simulink model "rlflight"  (R2024a)
settings: Solver=ode45  StartTime=0.0  StopTime=inf  RelTol=1e-3  EnableMultiTasking=on
libraries: instrumentlib x3, rllib x1
settings Model: Creator=The MathWorks, Inc.  LastModifiedBy=Administrator
settings SolverCC: AlgebraicLoopSolver=TrustRegion
settings DataIOCC: LimitDataPoints=on  SaveFormat=Array  SignalLoggingName=logsOut
settings OptimizationCC: ReuseModelBlockBuffer=off  ExpressionDepthLimit=2147483647  InitFltsAndDblsToZero=on  LifeSpan=inf
settings DebuggingCC: SaveWithParameterizedLinksMsg=none  UnderspecifiedInitializationDetection=Classic  MergeDetectMultiDrivingBlocksExec=none  SignalResolutionControl=TryResolveAllWithWarning  MultiTaskDSMMsg=warning  FcnCallInpInsideContextMsg=warning  UnconnectedInputMsg=warning  UnconnectedOutputMsg=warning  UnconnectedLineMsg=warning  AllowSymbolicDim=off  StateNameClashWarn=warning  SFUnexpectedBacktrackingDiag=warning  SFNoUnconditionalDefaultTransitionDiag=warning  SFExecutionAtInitializationDiag=none  ArithmeticOperatorsInVariantConditions=warning
settings HardwareCC: ProdBitPerPointer=32  ProdBitPerSizeT=32  ProdBitPerPtrDiffT=32  ProdLargestAtomicFloat=None  ProdIntDivRoundTo=Undefined  ProdEndianess=Unspecified  ProdWordSize=32  ProdHWDeviceType=Specified
settings ModelReferenceCC: EnableRefExpFcnMdlSchedulingChecks=on  PropagateSignalLabelsOutOfModel=off
settings SFSimCC: SimUseLocalCustomCode=off  CustomCodeUndefinedFunction=UseInterfaceOnly
settings RTWCC: RTWUseLocalCustomCode=off  GPUComputeCapability=3.5  DLArmComputeVersion=19.05
settings CodeAppCC: StateflowObjectComments=on
settings GRTTargetCC: TargetFcnLib=ansi_tfl_tmw.mat  TargetLangStandard=C89/C90 (ANSI)  CombineOutputUpdateFcns=off  GRTInterface=on
settings ConfigComp: CovMetricSettings=dw  CovSaveCumulativeToWorkspaceVar=on  CovSaveSingleToWorkspaceVar=on  CovExternalEMLEnable=off

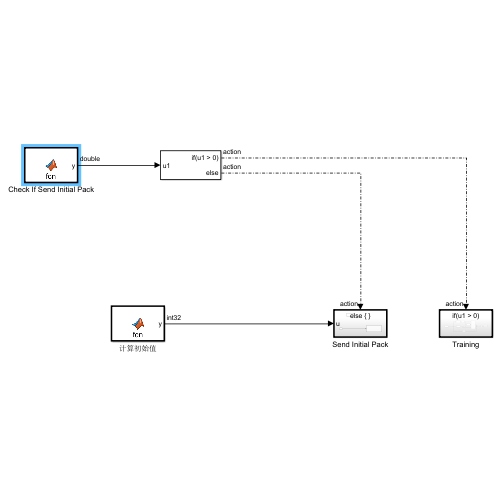
[thumbnail: Simulink's stored preview of the top-level diagram]
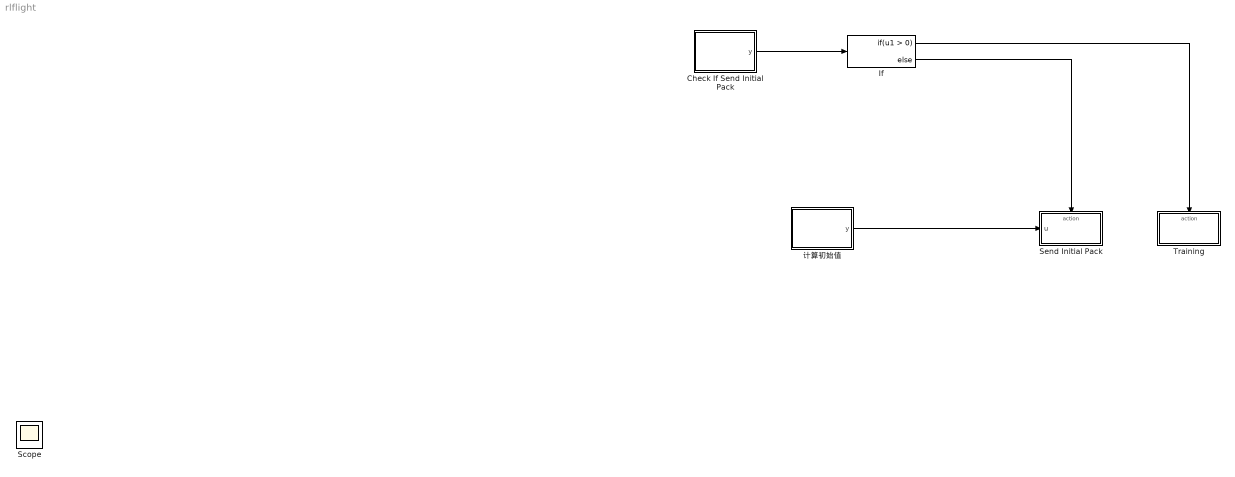
== system rlflight ==
  Check If Send Initial Pack : MATLAB Function  TreatAsAtomicUnit=on
  If : If
  Send Initial Pack : Subsystem  TreatAsAtomicUnit=on
  Training : Subsystem  TreatAsAtomicUnit=on
  计算初始值 : MATLAB Function  TreatAsAtomicUnit=on
  Scope : Scope
  wires:
  Check If Send Initial Pack/1(y) -> If/1
  If/2 -> Send Initial Pack/Action
  If/1 -> Training/Action
  计算初始值/1(y) -> Send Initial Pack/1(u)

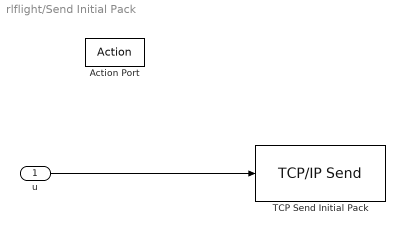
== system rlflight/Send Initial Pack ==
  u : Inport
  Action Port : ActionPort  ActionPortLabel=else
  TCP Send Initial Pack : instrumentlib/TCP//IP Send  Priority=1  Host=10.119.13.38  Port=1000  ByteOrder=little-endian  EnableBlockingMode=on  Timeout=5  TransferDelay=on  SimulateUsing=Interpreted execution
  wires:
  u/1 -> TCP Send Initial Pack/1

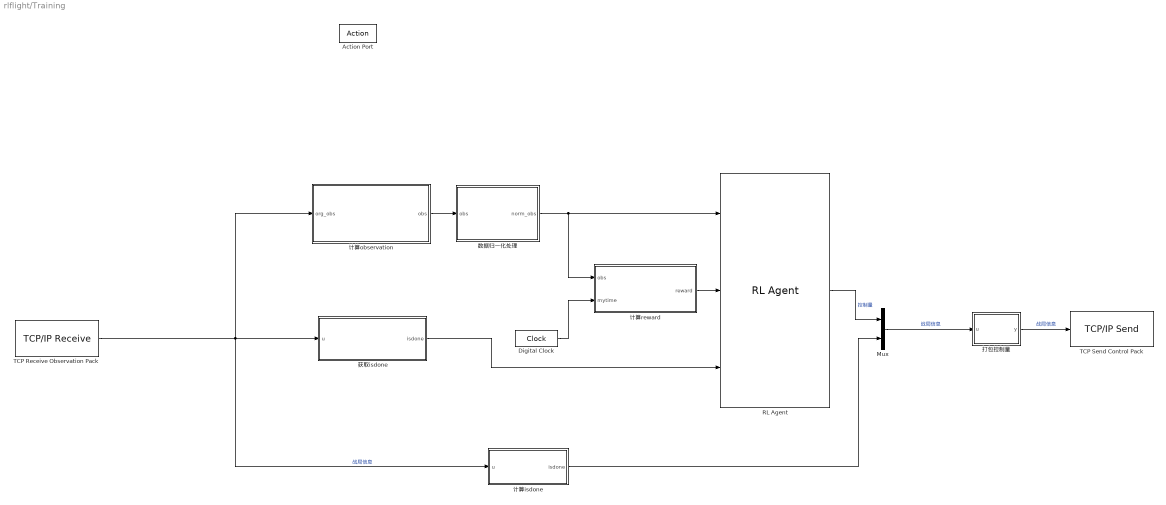
== system rlflight/Training ==
  Action Port : ActionPort  ActionPortLabel=if(u1 > 0)
  Digital Clock : DigitalClock
  Mux : Mux  Inputs=2
  RL Agent : rllib/RL Agent  Agent=agent  ExternalActionAsInput=off  ProvideLastAction=off  ProvideCumRwd=off  TreatAsDirectFeedthrough=on  UseStrictObservationDataTypes=off
  TCP Receive Observation Pack : instrumentlib/TCP//IP Receive  Priority=2  Host=10.119.13.38  Port=1000  DataSize=[ 1, 27 ]  DataType=double  ASCIIFormatting=%f  Terminator=LF  CustomTerminator=10  ByteOrder=little-endian  EnableBlockingMode=on  Timeout=20  SampleTime=-1  SimulateUsing=Interpreted execution
  TCP Send Control Pack : instrumentlib/TCP//IP Send  Priority=3  Host=10.119.13.38  Port=1000  ByteOrder=little-endian  EnableBlockingMode=on  Timeout=20  TransferDelay=off  SimulateUsing=Interpreted execution
  打包控制量 : MATLAB Function  TreatAsAtomicUnit=on
  数据归一化处理 : MATLAB Function  TreatAsAtomicUnit=on
  获取isdone : MATLAB Function  TreatAsAtomicUnit=on
  计算isdone : MATLAB Function  TreatAsAtomicUnit=on
  计算observation : MATLAB Function  TreatAsAtomicUnit=on
  计算reward : MATLAB Function  TreatAsAtomicUnit=on
  wires:
  计算reward/1(reward) -> RL Agent/2
  获取isdone/1(isdone) -> RL Agent/3
  数据归一化处理/1(norm_obs) -> 计算reward/1(obs), RL Agent/1
  计算isdone/1(isdone) -> Mux/2
  打包控制量/1(y) -> TCP Send Control Pack/1  "战局信息"
  TCP Receive Observation Pack/1 -> 计算isdone/1(u), 计算observation/1(org_obs), 获取isdone/1(u)  "战局信息"
  Digital Clock/1 -> 计算reward/2(mytime)
  RL Agent/1 -> Mux/1  "控制量"
  Mux/1 -> 打包控制量/1(u)  "战局信息"
  计算observation/1(obs) -> 数据归一化处理/1(obs)

== matlab function rlflight/Training/获取isdone ==
  data: u input; isdone output
function isdone = fcn(u)
isdone = u(27);
end

== matlab function rlflight/Training/计算reward ==
  data: obs input; reward output; mytime input
function reward = fcn(obs,mytime)
persistent pre_obs;
if isempty(pre_obs)
    pre_obs = obs;
end

% reward = get_tracking_reward(obs, pre_obs);
reward = get_my_reward(obs, pre_obs,mytime);

pre_obs = obs;
% if(abs(reward) > 100)
%     fprintf('reward = ');
%     disp(reward);
%     fprintf('\n');
% end
end

== matlab function rlflight/Training/计算observation ==
  data: org_obs input; obs output
function obs = fcn(org_obs)
% obs = get_tracking_obs(org_obs);
obs = get_my_obs(org_obs);
end

== matlab function rlflight/Training/数据归一化处理 ==
  data: obs input; norm_obs output
function norm_obs = fcn(obs)
norm_obs = normalize_my_obs(obs);
end

== matlab function rlflight/Training/计算isdone ==
  data: u input; isdone output double size=1
function isdone = fcn(u)
isdone = get_my_isdone(u);
end

== matlab function rlflight/Check If Send Initial Pack ==
  data: y output
function y = fcn()
%判断是否为第一个回合
persistent ifSendInitPack;
if isempty(ifSendInitPack)
    ifSendInitPack = 0;
end
y = ifSendInitPack;
if(ifSendInitPack == 0)
    ifSendInitPack = 1;
end
end

== matlab function rlflight/计算初始值 ==
  data: y output
function y = fcn()
y = get_my_initial();
end

== matlab function rlflight/Training/打包控制量 ==
  data: u input; y output
function y = fcn(u)
   % 打包成数组供TCP模块发送到服务器
   % 通信协议如下
   % [throttle，pitch，roll，yaw，is_done]
   % 根据obs与act中的配置，不让智能体控制滚转，只通过油门、俯仰、偏航三个控制量进行控制
   y = [u(1), u(2), 0, u(3), u(4)];
